simulink library "Generator_Lib"  (R2025a)
settings: Solver=ode45  StartTime=0.0  StopTime=10.0  RelTol=1e-3  EnableMultiTasking=on
undefined symbols (not defined in the file or in its folder): DiscIntNeverNeededParam, K, Lambda, radps2rpm, tau, WT_Params, x0
libraries: fl_lib x24, nesl_utility x16, ee_lib x14, simulink x1
(part 1 of 2)
Description:
  | Copyright 2009-2024 The MathWorks, Inc. MathWorks, Inc.
settings Model: Creator=smiller  LastModifiedBy=smiller
settings SolverCC: AlgebraicLoopSolver=TrustRegion
settings DataIOCC: LimitDataPoints=on  SaveFormat=Array  SignalLoggingSaveFormat=ModelDataLogs  ReturnWorkspaceOutputs=off
settings OptimizationCC: ReuseModelBlockBuffer=off  ExpressionDepthLimit=2147483647.0  LifeSpan=inf
settings DebuggingCC: UnderspecifiedInitializationDetection=Classic  MergeDetectMultiDrivingBlocksExec=none  SolverPrmCheckMsg=warning  FcnCallInpInsideContextMsg=warning  UnconnectedInputMsg=warning  UnconnectedOutputMsg=warning  UnconnectedLineMsg=warning  AllowSymbolicDim=off  StateNameClashWarn=warning  PregeneratedLibrarySubsystemCodeDiagnostic=none  SFUnexpectedBacktrackingDiag=warning  SFNoUnconditionalDefaultTransitionDiag=warning  SFExecutionAtInitializationDiag=none  ArithmeticOperatorsInVariantConditions=warning
settings HardwareCC: ProdBitPerPointer=32.0  ProdBitPerSizeT=32.0  ProdBitPerPtrDiffT=32.0  ProdLargestAtomicFloat=None  ProdIntDivRoundTo=Undefined  ProdEndianess=Unspecified  ProdWordSize=32.0  ProdHWDeviceType=32-bit Generic
settings ModelReferenceCC: EnableRefExpFcnMdlSchedulingChecks=on  PropagateSignalLabelsOutOfModel=off
settings SFSimCC: SimUseLocalCustomCode=off  CustomCodeUndefinedFunction=UseInterfaceOnly
settings RTWCC: RTWUseLocalCustomCode=off  GPUComputeCapability=3.5  DLArmComputeVersion=19.05
settings CodeAppCC: StateflowObjectComments=on
settings GRTTargetCC: TargetLangStandard=C89/C90 (ANSI)  CombineOutputUpdateFcns=off  GRTInterface=on
settings ConfigComp: CovMetricSettings=dw  CovSaveCumulativeToWorkspaceVar=on  CovSaveSingleToWorkspaceVar=on  CovExternalEMLEnable=off  CovSFcnEnable=off

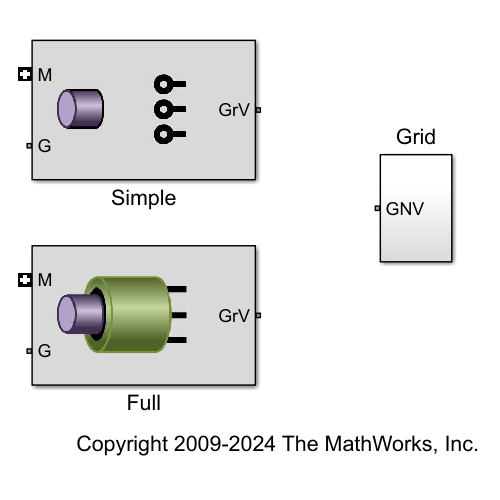
[thumbnail: Simulink's stored preview of the top-level diagram]
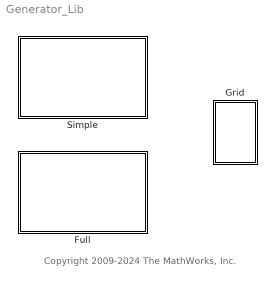
== system Generator_Lib ==
  note: Copyright 2009-2024 The MathWorks, Inc.
  Full : Subsystem  VariantControl=Full
      mask Display: image('Generator_Full_IMAGE.jpg');
  Grid : Subsystem
  Simple : Subsystem  VariantControl=Simple
      mask Display: image('Generator_Simple_IMAGE.jpg');

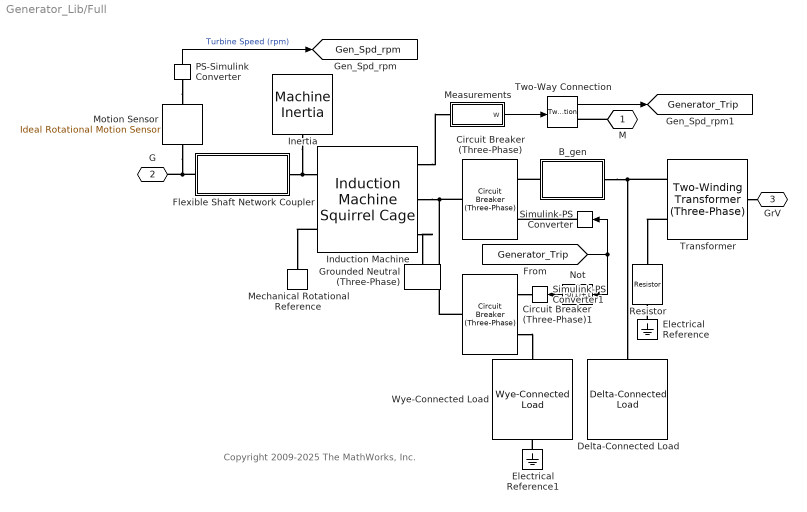
== system Generator_Lib/Full ==
  note: Copyright 2009-2025 The MathWorks, Inc.
  "B_gen " : Subsystem  mask{volt_meas=Phase-to-Ground (Phase Voltage), meas_units=PU, Vnom=WT_Params.Generator.voltage, Pnom=WT_Params.Generator.nominal_power}
      mask prompts: volt_meas "Voltage Measurement"; meas_units "Measurement Units"; Vnom "Nominal Voltage (Vrms)"; Pnom "Nominal Power (VA)"
      mask init:
      | volt_meas  = get_param(gcb,'volt_meas');
      | meas_units = get_param(gcb,'meas_units');
      | 
      | path_CV = [gcb,'/current_voltage'];
      | 
      | switch volt_meas
      | 
      |     case 'Phase-to-Ground (Phase Voltage)'
      | 
      |         set_param(path_CV,'vMeasurementType','ee.enum.vmeasurement.lg')
      | 
      |     case 'Line-to-Line (Line Voltage)'
      | 
      |         set_param(path_CV,'vMeasurementType','ee.enum.vmeasurement.ll')
      | 
      | end
      | 
      | switch meas_units
      | 
      |     case 'SI'
      | 
      |         set_param(path_CV,'outputUnit','ee.enum.unit.si')
      |         
      | 
      |     case 'PU'
      | 
      |         set_param(path_CV,'outputUnit','ee.enum.unit.pu')
      |       
      | 
      | end
      mask TypeOptions volt_meas: Phase-to-Ground (Phase Voltage) | Line-to-Line (Line Voltage)
      mask TypeOptions meas_units: SI | PU
      mask Callback meas_units:
      | meas_units = get_param(gcb,'meas_units');
      | 
      | switch meas_units
      | 
      |     case 'SI'
      | 
      |         set_param(gcb,'MaskVisibilities',{'on','on','off','off'})
      | 
      | 
      |     case 'PU'
      | 
      |         set_param(gcb,'MaskVisibilities',{'on','on','on','on'})
      | 
      | 
      | end
      mask DialogControl Container1 Prompt: Voltage and Current Measurement
      mask DialogControl Container2 Prompt: The block represents an ideal three-phase voltage and current sensor.
  Circuit Breaker (Three-Phase) : ee_lib/Switches & Breakers/Circuit Breaker (Three-Phase)  R_closed=WT_Params.Generator.Breakers.ron Ohm  G_open=1/WT_Params.Generator.Breakers.rp 1/Ohm  threshold=0.5 V  breaker_behavior=ee.enum.switches.breakerBehavior.zeroCrossingEnable
      settings: InternalSimscapePortConfiguration="{\"Bottom\":[],\"Left\":[{\"id\":\"vT\",\"label\":\"vT\",\"type\":\"input\"},{\"id\":\"N1\",\"label\":\"~1\",\"type\":\"foundation.electrical.three_phase\"}],\"Right\":[{\"id\":\"N2\",\"label\":\"~2\",\"type\":\"foundation.electrical.three_phase\"}],\"Top\":[]}"
  Circuit Breaker (Three-Phase)1 : ee_lib/Switches & Breakers/Circuit Breaker (Three-Phase)  R_closed=WT_Params.Generator.Breakers.ron Ohm  G_open=1/WT_Params.Generator.Breakers.rp 1/Ohm  threshold=0.5 V  breaker_behavior=ee.enum.switches.breakerBehavior.zeroCrossingEnable
      settings: InternalSimscapePortConfiguration="{\"Bottom\":[],\"Left\":[{\"id\":\"vT\",\"label\":\"vT\",\"type\":\"input\"},{\"id\":\"N1\",\"label\":\"~1\",\"type\":\"foundation.electrical.three_phase\"}],\"Right\":[{\"id\":\"N2\",\"label\":\"~2\",\"type\":\"foundation.electrical.three_phase\"}],\"Top\":[]}"
  Delta-Connected Load : ee_lib/Passive/RLC Assemblies/Delta-Connected Load  port_option=ee.enum.threePhasePort.composite  parameterization=ee.enum.rlc.parameterization.ratedpower  component_structure=ee.enum.rlc.structure.R  component_structure_PQ=ee.enum.rlc.structure.C  R=1 Ohm  L=1e-3 H  C=1e-6 F  VRated=WT_Params.Generator.voltage V  FRated=WT_Params.Generator.frequency Hz  P=1e3 W  Qpos=1e2 A*V  Qneg=-200e3 A*V  R_parasitic=0 Ohm  G_parasitic=0 1/Ohm  R_parasitic_PQ=0 Ohm  G_parasitic_PQ=0 1/Ohm  Vmag0=24e3 V  Vang0=0 deg  Freq0=60 Hz  IL_specify=off  IL_priority=High  IL=[0, 0, 0] A  IL_nominal_specify=off  IL_nominal_value=1  IL_nominal_unit=A  VC_specify=off  VC_priority=High  VC=[0, 0, 0] V  VC_nominal_specify=off  VC_nominal_value=1  VC_nominal_unit=V
      settings: InternalSimscapePortConfiguration="{\"Bottom\":[],\"Left\":[{\"id\":\"N\",\"label\":\"~\",\"type\":\"foundation.electrical.three_phase\"}],\"Right\":[],\"Top\":[]}"
  Electrical Reference : fl_lib/Electrical/Electrical Elements/Electrical Reference
  Electrical Reference1 : fl_lib/Electrical/Electrical Elements/Electrical Reference
  Flexible Shaft Network Coupler : Subsystem  mask(Network Coupler (Flexible Shaft)){}
      mask init:
      | % Icon
      | key = 'Simscape.NetworkCouplers.FlexibleShaft';
      | foundation.internal.couplers.updateIcon(gcb,'flexibleShaft.svg',key)
      settings: OpenFcn=open_system(gcbh,'force')
      mask Help: web([docroot '/simscape/ref/networkcouplerflexibleshaft.html'])
      mask Display:
      | color('red');
      | port_label('LConn', 1,'1')
      | port_label('RConn', 1,'2')
  Grounded Neutral (Three-Phase) : ee_lib/Connectors & References/Grounded Neutral (Three-Phase)
  Induction Machine : ee_lib/Electromechanical/Asynchronous/Induction Machine Squirrel Cage  port_option=ee.enum.threePhasePort.composite  SRated=WT_Params.Generator.nominal_power A*V  VRated=WT_Params.Generator.voltage V  FRated=WT_Params.Generator.frequency Hz  nPolePairs=3  param_unit=ee.enum.unit.pu  squirrel_cage=ee.enum.squirrelcage.Single  zero_sequence=ee.enum.park.zerosequence.exclude  initialization_option=ee.enum.asm.initialization.fluxvariables  Rs=Rs Ohm  Xls=Xls Ohm  pu_Rs=WT_Params.Generator.Stator.resistance  pu_Lls=WT_Params.Generator.Stator.inductance  Rrd=Rrp Ohm  Xlrd=Xlrp Ohm  pu_Rrd=WT_Params.Generator.Rotor.resistance  pu_Llrd=WT_Params.Generator.Rotor.inductance  Rrd1=0.28 Ohm  Xlrd1=0.82 Ohm  Rrd2=0.28 Ohm  Xlrd2=0.82 Ohm  pu_Rrd1=0.0290  pu_Llrd1=0.0848  pu_Rrd2=0.0290  pu_Llrd2=0.0848  Xm=Xm Ohm  pu_Lm=WT_Params.Generator.mutual_inductance  X0=0.4 Ohm  pu_L0=0.0413  saturation_option=ee.enum.saturation.exclude  saturation_i=[0, 4, 9, 18, 25, 34, 50, 68, 95, 120] A  saturation_v=[0, 88, 154, 198, 220, 242, 264, 286, 308, 327] V  pu_saturation_i=[0, .176, .396, .792, 1.1, 1.496, 2.2, 2.992, 4.18, 5.28]  pu_saturation_v=[0, .4, .7, .9, 1, 1.1, 1.2, 1.3, 1.4, 1.4864]  connection_option=ee.enum.Connection.delta  angular_position_specify=off  angular_position_priority=None  angular_position=0 deg  angular_position_nominal_specify=off  angular_position_nominal_value=1  angular_position_nominal_unit=deg  pu_psids_specify=off  pu_psids_priority=None  pu_psids=0  pu_psids_nominal_specify=off  pu_psids_nominal_value=1  pu_psids_nominal_unit=1  pu_psiqs_specify=off  pu_psiqs_priority=None  pu_psiqs=0  pu_psiqs_nominal_specify=off  pu_psiqs_nominal_value=1  pu_psiqs_nominal_unit=1  pu_psi0s_specify=off  pu_psi0s_priority=None  pu_psi0s=0  pu_psi0s_nominal_specify=off  pu_psi0s_nominal_value=1  pu_psi0s_nominal_unit=1  pu_psidr_specify=off  pu_psidr_priority=None  pu_psidr=0  pu_psidr_nominal_specify=off  pu_psidr_nominal_value=1  pu_psidr_nominal_unit=1  pu_psiqr_specify=off  pu_psiqr_priority=None  pu_psiqr=0  pu_psiqr_nominal_specify=off  pu_psiqr_nominal_value=1  pu_psiqr_nominal_unit=1  pu_psidr1_specify=off  pu_psidr1_priority=None  pu_psidr1=0  pu_psidr1_nominal_specify=off  pu_psidr1_nominal_value=1  pu_psidr1_nominal_unit=1  pu_psiqr1_specify=off  pu_psiqr1_priority=None  pu_psiqr1=0  pu_psiqr1_nominal_specify=off  pu_psiqr1_nominal_value=1  pu_psiqr1_nominal_unit=1  pu_psidr2_specify=off  pu_psidr2_priority=None  pu_psidr2=0  pu_psidr2_nominal_specify=off  pu_psidr2_nominal_value=1  pu_psidr2_nominal_unit=1  pu_psiqr2_specify=off  pu_psiqr2_priority=None  pu_psiqr2=0  pu_psiqr2_nominal_specify=off  pu_psiqr2_nominal_value=1  pu_psiqr2_nominal_unit=1  psids_specify=off  psids_priority=None  psids=0 Wb  psids_nominal_specify=off  psids_nominal_value=1  psids_nominal_unit=Wb  psiqs_specify=off  psiqs_priority=None  psiqs=0 Wb  psiqs_nominal_specify=off  psiqs_nominal_value=1  psiqs_nominal_unit=Wb  psi0s_specify=off  psi0s_priority=None  psi0s=0 Wb  psi0s_nominal_specify=off  psi0s_nominal_value=1  psi0s_nominal_unit=Wb  psidr_specify=off  psidr_priority=None  psidr=0 Wb  psidr_nominal_specify=off  psidr_nominal_value=1  psidr_nominal_unit=Wb  psiqr_specify=off  psiqr_priority=None  psiqr=0 Wb  psiqr_nominal_specify=off  psiqr_nominal_value=1  psiqr_nominal_unit=Wb  psidr1_specify=off  psidr1_priority=None  psidr1=0 Wb  psidr1_nominal_specify=off  psidr1_nominal_value=1  psidr1_nominal_unit=Wb  psiqr1_specify=off  psiqr1_priority=None  psiqr1=0 Wb  psiqr1_nominal_specify=off  psiqr1_nominal_value=1  psiqr1_nominal_unit=Wb  psidr2_specify=off  psidr2_priority=None  psidr2=0 Wb  psidr2_nominal_specify=off  psidr2_nominal_value=1  psidr2_nominal_unit=Wb  psiqr2_specify=off  psiqr2_priority=None  psiqr2=0 Wb  psiqr2_nominal_specify=off  psiqr2_nominal_value=1  psiqr2_nominal_unit=Wb  slip_specify=off  slip_priority=None  slip=0  slip_nominal_specify=off  slip_nominal_value=1  slip_nominal_unit=1  real_power_generated_specify=off  real_power_generated_priority=None  real_power_generated=0 W  real_power_generated_nominal_specify=off  real_power_generated_nominal_value=1  real_power_generated_nominal_unit=W  mechanical_power_consumed_specify=off  mechanical_power_consumed_priority=None  mechanical_power_consumed=0 W  mechanical_power_consumed_nominal_specify=off  mechanical_power_consumed_nominal_value=1  mechanical_power_consumed_nominal_unit=W  Tmeas=298.15 K  alpha=3.93e-3 1/K  alpha_cage=4.4e-3 1/K  stator_thermal_mass=100 J/K  rotor_thermal_mass=200 J/K  temperatureA_specify=off  temperatureA_priority=High  temperatureA=25 degC  temperatureA_nominal_specify=off  temperatureA_nominal_value=1  temperatureA_nominal_unit=degC  temperatureB_specify=off  temperatureB_priority=High  temperatureB=25 degC  temperatureB_nominal_specify=off  temperatureB_nominal_value=1  temperatureB_nominal_unit=degC  temperatureC_specify=off  temperatureC_priority=High  temperatureC=25 degC  temperatureC_nominal_specify=off  temperatureC_nominal_value=1  temperatureC_nominal_unit=degC  temperatureR_specify=off  temperatureR_priority=High  temperatureR=25 degC  temperatureR_nominal_specify=off  temperatureR_nominal_value=1  temperatureR_nominal_unit=degC
      settings: InternalSimscapePortConfiguration="{\"Bottom\":[],\"Left\":[{\"id\":\"R\",\"label\":\"R\",\"type\":\"foundation.mechanical.rotational.rotational\"},{\"id\":\"C\",\"label\":\"C\",\"type\":\"foundation.mechanical.rotational.rotational\"}],\"Right\":[{\"id\":\"pu_output\",\"label\":\"pu\",\"type\":\"output\"},{\"id\":\"N1\",\"label\":\"~1\",\"type\":\"foundation.electrical.three_phase\"},{\"id\":\"N2\",\"label\":\"~2\",\"type\":\"foundation.electrical.three_phase\"}],\"Top\":[]}"
  Inertia : ee_lib/Electromechanical/Mechanical/Machine Inertia  SRated=WT_Params.Generator.nominal_power A*V  FRated=WT_Params.Generator.frequency Hz  nPolePairs=3  inertia_option=1  J=3 kg*m^2  H=3.525 W*s/(A*V)  damper_option=2  D=39.0509 N*m*s/rad  pu_D=0  initialization_option=2  fMechanical0=60 Hz  fElectrical0=0 Hz
      settings: InternalSimscapePortConfiguration="{\"Bottom\":[],\"Left\":[{\"id\":\"R\",\"label\":\"R\",\"type\":\"foundation.mechanical.rotational.rotational\"}],\"Right\":[],\"Top\":[]}"
  Measurements : Subsystem
  Mechanical Rotational Reference : fl_lib/Mechanical/Rotational Elements/Mechanical Rotational Reference
  Motion Sensor : fl_lib/Mechanical/Mechanical Sensors/Ideal Rotational Motion Sensor  reference=foundation.enum.MeasurementReference.absolute  acceleration_port=false  velocity_port=true  position_port=false  wrap_angle=simscape.enum.onoff.off  offset=0 rad
      settings: InternalSimscapePortConfiguration="{\"Bottom\":[],\"Left\":[{\"id\":\"R\",\"label\":\"R\",\"type\":\"foundation.mechanical.rotational.rotational\"}],\"Right\":[{\"id\":\"W\",\"label\":\"W\",\"type\":\"output\"}],\"Top\":[]}"
  Not : Fcn  Expr=-u(1)+1
  PS-Simulink Converter : nesl_utility/PS-Simulink Converter  PhysicalDomain=network_engine_domain  SubClassName=ps_output  LeftPortType=input  RightPortType=output  PseudoPeriodic=off  Frequencies=[]  VectorFormat=1-D array  Unit=rpm  AffineConversion=off
  Resistor : fl_lib/Electrical/Electrical Elements/Resistor  R=10 Ohm  i_specify=off  i_priority=None  i=0 A  i_nominal_specify=off  i_nominal_value=1  i_nominal_unit=A  v_specify=off  v_priority=None  v=0 V  v_nominal_specify=off  v_nominal_value=1  v_nominal_unit=V
  Simulink-PS Converter : nesl_utility/Simulink-PS Converter  PhysicalDomain=network_engine_domain  SubClassName=ps_input  LeftPortType=input  RightPortType=output  PseudoPeriodic=off  Frequencies=[]  NoiseDistribution=none  NoiseParameters=[]  Unit=1  AffineConversion=off  FilteringAndDerivatives=provide  SimscapeFilterOrder=1  InputFilterTimeConstant=0.001  UdotUserProvided=0
  Simulink-PS Converter1 : nesl_utility/Simulink-PS Converter  PhysicalDomain=network_engine_domain  SubClassName=ps_input  LeftPortType=input  RightPortType=output  PseudoPeriodic=off  Frequencies=[]  NoiseDistribution=none  NoiseParameters=[]  Unit=1  AffineConversion=off  FilteringAndDerivatives=provide  SimscapeFilterOrder=1  InputFilterTimeConstant=0.001  UdotUserProvided=0
  Transformer : ee_lib/Passive/Transformers/Two-Winding Transformer (Three-Phase)  SRated=2e6 A*V  FRated=60 Hz  Winding1Connection=ee.enum.windingconnection.Yg  VRated1=WT_Params.Grid.voltage V  Winding2Connection=ee.enum.windingconnection.Yn  VRated2=WT_Params.Generator.voltage V  CoreType=ee.enum.coretype.threelimb  pu_Rw1=0.025/30  pu_Rw2=0.025/30  leakage_reactance_option=ee.enum.transformer_leakage.include  pu_Xl1=0.025  pu_Xl2=0.025  magnetizing_resistance_option=ee.enum.transformer_magnetizingResistance.include  pu_Rm=500  magnetizing_reactance_option=ee.enum.transformer_magnetizingReactance.include  saturation_option=ee.enum.transformer_saturation.exclude  pu_Xm=500  current_data=[0, .002, 1, 2]  magnetic_flux_data=[0, 1.2, 1.5, 1.51]  pu_X0=0.5  i1_specify=off  i1_priority=None  i1=[0, 0, 0] A  i1_nominal_specify=off  i1_nominal_value=1  i1_nominal_unit=A  i2_specify=off  i2_priority=None  i2=[0, 0, 0] A  i2_nominal_specify=off  i2_nominal_value=1  i2_nominal_unit=A  phi_specify=off  phi_priority=None  phi=[0, 0, 0]  phi_nominal_specify=off  phi_nominal_value=1  phi_nominal_unit=1  power_dissipated_specify=off  power_dissipated_priority=None  power_dissipated=0 W  power_dissipated_nominal_specify=off  power_dissipated_nominal_value=1  power_dissipated_nominal_unit=W
      settings: InternalSimscapePortConfiguration="{\"Bottom\":[],\"Left\":[{\"id\":\"N1\",\"label\":\"~1\",\"type\":\"foundation.electrical.three_phase\"}],\"Right\":[{\"id\":\"N2\",\"label\":\"~2\",\"type\":\"foundation.electrical.three_phase\"},{\"id\":\"n2\",\"label\":\"n2\",\"type\":\"foundation.electrical.electrical\"}],\"Top\":[]}"
  Two-Way Connection : TwoWayConnection
  Wye-Connected Load : ee_lib/Passive/RLC Assemblies/Wye-Connected Load  port_option=ee.enum.threePhasePort.composite  parameterization=ee.enum.rlc.parameterization.ratedpower  component_structure=ee.enum.rlc.structure.R  component_structure_PQ=ee.enum.rlc.structure.R  R=1 Ohm  L=1e-3 H  C=1e-6 F  VRated=WT_Params.Generator.voltage V  FRated=60 Hz  P=WT_Params.Generator.nominal_power W  Qpos=1e2 A*V  Qneg=-1e2 A*V  R_parasitic=0 Ohm  G_parasitic=0 1/Ohm  R_parasitic_PQ=0 Ohm  G_parasitic_PQ=0 1/Ohm  Vmag0=24e3 V  Vang0=0 deg  Freq0=60 Hz  IL_specify=off  IL_priority=High  IL=[0, 0, 0] A  IL_nominal_specify=off  IL_nominal_value=1  IL_nominal_unit=A  VC_specify=off  VC_priority=High  VC=[0, 0, 0] V  VC_nominal_specify=off  VC_nominal_value=1  VC_nominal_unit=V
  M : PMIOPort  Tag=PMCPort  Side=Left
  G : PMIOPort  Port=2  Side=Left
  GrV : PMIOPort  Port=3  Side=Right
  tag scope: Gen_Spd_rpm=global, Generator_Trip=global
  wires:
  PS-Simulink Converter/1 -> [Gen_Spd_rpm]  "Turbine Speed (rpm)"
  Two-Way Connection/1 -> [Generator_Trip]
  Not/1 -> Simulink-PS Converter1/1
  [Generator_Trip] -> Not/1, Simulink-PS Converter/1
  Measurements/1(w) -> Two-Way Connection/1
  connections:
  Flexible Shaft Network Coupler/LConn1 -- G/RConn1 -- Motion Sensor/LConn1
  M/RConn1 -- Two-Way Connection/RConn1
  Transformer/LConn1 -- GrV/RConn1
  Electrical Reference/LConn1 -- Resistor/LConn1
  Transformer/RConn2 -- Resistor/RConn1
  Transformer/RConn1 -- "B_gen "/RConn1 -- Delta-Connected Load/LConn1
  Circuit Breaker (Three-Phase)/RConn1 -- Circuit Breaker (Three-Phase)1/RConn1 -- Induction Machine/RConn2
  Electrical Reference1/LConn1 -- Wye-Connected Load/RConn1
  "B_gen "/LConn1 -- Circuit Breaker (Three-Phase)/LConn2
  Circuit Breaker (Three-Phase)1/LConn2 -- Wye-Connected Load/LConn1
  Simulink-PS Converter/RConn1 -- Circuit Breaker (Three-Phase)/LConn1
  Circuit Breaker (Three-Phase)1/LConn1 -- Simulink-PS Converter1/RConn1
  PS-Simulink Converter/LConn1 -- Motion Sensor/RConn1
  Induction Machine/LConn2 -- Mechanical Rotational Reference/LConn1
  Flexible Shaft Network Coupler/RConn1 -- Inertia/LConn1 -- Induction Machine/LConn1
  Induction Machine/RConn3 -- Grounded Neutral (Three-Phase)/LConn1
  Induction Machine/RConn1 -- Measurements/LConn1

== system Generator_Lib/Grid ==
  note: Copyright 2009-2025 The MathWorks, Inc.
  Electrical Reference : fl_lib/Electrical/Electrical Elements/Electrical Reference
  Grid : ee_lib/Sources/Voltage Source (Three-Phase)  vline_rms=WT_Params.Grid.voltage V  shift=0 deg  freq=WT_Params.Grid.frequency Hz  impedance_option=0  SShortCircuit=1e6 A*V  XR=15  R=0.01 Ohm  L=3.97e-4 H  harmonic_option=0  harmonic_orders=[5, 7, 11, 13]  harmonic_ratios=[.1, .1, .1, .1]  G_parasitic=0 1/Ohm  I_specify=off  I_priority=None  I=[0, 0, 0] A  I_nominal_specify=off  I_nominal_value=1  I_nominal_unit=A
  Mutual RL Pos-Zero (SI) : Subsystem  mask{R1_L1=[0.1  1.0/(2*pi*60)]*WT_Params.Grid.voltage^2/2500e6, R0_L0=[0.3  3.0/(2*pi*60)]*WT_Params.Grid.voltage^2/2500e6, run_time=off}
      mask prompts: R1_L1 "Positive Sequence [R1(Ohm) L1(H)]"; R0_L0 "Zero Sequence [R0(Ohm) L0(H)]"; run_time "Set parameters to run-time (model does not recompile if parameters change value)"
      mask init:
      | maskObj = Simulink.Mask.get(gcbh);
      | workspaceObj = maskObj.getWorkspace();
      | 
      | R1_L1 = workspaceObj.get('R1_L1');
      | R0_L0 = workspaceObj.get('R0_L0');
      | 
      | R1_si = R1_L1(1);
      | L1_si = R1_L1(2);
      | R0_si = R0_L0(1);
      | L0_si = R0_L0(2);
      | 
      | Rs_si = (2*R1_si + R0_si)/3;
      | Rm_si = (R0_si - R1_si)/3;
      | 
      | Ls_si = (2*L1_si + L0_si)/3;
      | Lm_si = (L0_si - L1_si)/3;
      mask Callback run_time:
      | run_time = get_param(gcb,'run_time');
      | 
      | path_coupled = [gcb,'/Coupled'];
      | 
      | switch run_time
      |     case 'off'
      |         pcr = 'compiletime';
      |     case 'on'
      |         pcr = 'runtime';
      | end
      | 
      | set_param(path_coupled,'R_conf',pcr)
      | set_param(path_coupled,'Rm_conf',pcr)
      | set_param(path_coupled,'L_conf',pcr)
      | set_param(path_coupled,'Lm_conf',pcr)
      mask DialogControl DescGroupVar Prompt: Mutual RL Pos-Zero
      mask DialogControl DescTextVar Prompt: Define mutual RL with positive and zero sequence values
      mask DialogControl Container5 Prompt: Parameters
      mask Display: disp('Mutual RL\n Pos-Zero\n(SI)')
  Pi-Section Pos-Zero (SI) : Subsystem  mask{length=1, Fnom=WT_Params.Grid.frequency, R1_L1_C1=[0.1153 1.05e-3 11.33e-9], R0_L0_C0=[0.413 3.32e-3 5.01e-9], run_time=off}
      mask prompts: length "Line Length (km)"; Fnom "Nominal Frequency (Hz)"; R1_L1_C1 "Positive Sequence [R1(Ohm/km) L1(H/km) C1(F/km)]"; R0_L0_C0 "Zero Sequence [R0(Ohm/km) L0(H/km) C0(F/km)]"; run_time "Set parameters to run-time (model does not recompile if parameters change value)"
      mask init:
      | maskObj = Simulink.Mask.get(gcbh);
      | workspaceObj = maskObj.getWorkspace();
      | 
      | R1_L1_C1 = workspaceObj.get('R1_L1_C1');
      | R0_L0_C0 = workspaceObj.get('R0_L0_C0');
      | 
      | R1_si = R1_L1_C1(1);
      | L1_si = R1_L1_C1(2);
      | C1_si = R1_L1_C1(3);
      | R0_si = R0_L0_C0(1);
      | L0_si = R0_L0_C0(2);
      | C0_si = R0_L0_C0(3);
      | 
      | Rs_si = (2*R1_si + R0_si)/3;
      | Rm_si = (R0_si - R1_si)/3;
      | 
      | Ls_si = (2*L1_si + L0_si)/3;
      | Lm_si = (L0_si - L1_si)/3;
      | 
      | Cl_si = (C1_si-C0_si)/3;
      | Cg_si = C0_si;
      mask Callback run_time:
      | run_time = get_param(gcb,'run_time');
      | 
      | path_line = [gcb,'/line'];
      | 
      | switch run_time
      |     case 'off'
      |         pcr = 'compiletime';
      |     case 'on'
      |         pcr = 'runtime';
      | end
      | 
      | set_param(path_line,'freq_conf',pcr)
      | set_param(path_line,'length_conf',pcr)
      | set_param(path_line,'R_conf',pcr)
      | set_param(path_line,'L_conf',pcr)
      | set_param(path_line,'Rm_conf',pcr)
      | set_param(path_line,'M_conf',pcr)
      | set_param(path_line,'Cg_conf',pcr)
      | set_param(path_line,'Cl_conf',pcr)
      mask DialogControl DescGroupVar Prompt: Pi-Section Pos-Zero (SI)
      mask DialogControl DescTextVar Prompt: Define pi-section line with positive and zero sequence values
      mask DialogControl Container5 Prompt: Parameters
      mask Display: disp('Pi-Section\nPos-Zero\n(SI)')
  GNV : PMIOPort  Side=Right
  connections:
  Grid/RConn1 -- Mutual RL Pos-Zero (SI)/RConn1
  Electrical Reference/LConn1 -- Grid/LConn1
  Mutual RL Pos-Zero (SI)/LConn1 -- Pi-Section Pos-Zero (SI)/RConn1
  GNV/RConn1 -- Pi-Section Pos-Zero (SI)/LConn1

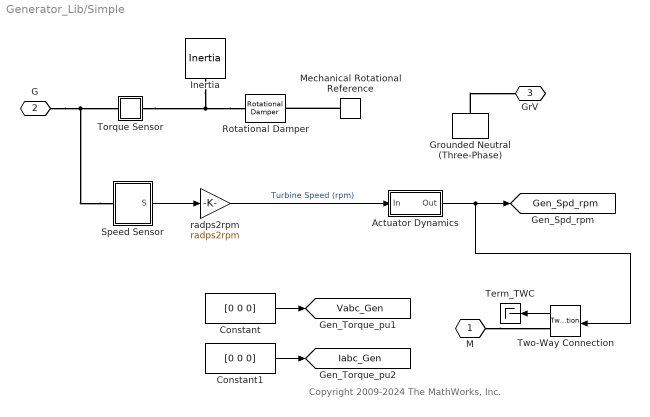
== system Generator_Lib/Simple ==
  note: Copyright 2009-2024 The MathWorks, Inc.
  Actuator Dynamics : Subsystem  mask(First-order lag supporting vector signals){b=WT_Params.Generator.generator_time_constant, x_initial=0}
      mask prompts: b "Filter time constant"; x_initial "Initial output"
      mask help: Models a lag of the form 1/(b*s+1) where s is the Laplace operator.
  Constant : Constant  Value=[0 0 0]  OutDataTypeStr=Inherit: Inherit via back propagation
  Constant1 : Constant  Value=[0 0 0]  OutDataTypeStr=Inherit: Inherit via back propagation
  Grounded Neutral (Three-Phase) : ee_lib/Connectors & References/Grounded Neutral (Three-Phase)
  Inertia : fl_lib/Mechanical/Rotational Elements/Inertia  inertia=WT_Params.Generator.Simple.inertia kg*m^2  num_ports=foundation.enum.numPorts2.one  w_specify=on  w_priority=High  w=0 rad/s  w_nominal_specify=off  w_nominal_value=1  w_nominal_unit=rad/s  t_specify=off  t_priority=High  t=0 N*m  t_nominal_specify=off  t_nominal_value=1  t_nominal_unit=N*m
  Mechanical Rotational Reference : fl_lib/Mechanical/Rotational Elements/Mechanical Rotational Reference
  Rotational Damper : fl_lib/Mechanical/Rotational Elements/Rotational Damper  D=WT_Params.Generator.Simple.damping N*m/(rad/s)  w_specify=off  w_priority=High  w=0 rad/s  w_nominal_specify=off  w_nominal_value=1  w_nominal_unit=rad/s  t_specify=off  t_priority=High  t=0 N*m  t_nominal_specify=off  t_nominal_value=1  t_nominal_unit=N*m
  Speed Sensor : Subsystem
      mask Display:
      | plot([149.600878633536;150.016472378793;150.47508104106;150.972287968219;151.50330478576;152.063017511447;152.646035805762;153.246744883819;153.859359588817;154.477980106257;155.096648782383;155.709407499646;156.310355056631;156.893703999851;157.453836360095;157.985357756531;158.483149347555;158.942417128023;159.358738098149;159.728102859405;160.046954227227;160.312221488639;160.521349974904;160.672325664379;160.763694578642;160.794576785101;160.764674871227;160.674276808796;160.524253180566;160.316048796087;160.051668777399;159.733659248606;159.365082815313;158.949489070056;158.490880407788;157.993673480629;157.462656663088;156.908284800231], [156.971389291536;157.430657072004;157.84697804213;158.216342803387;158.535194171208;158.80046143262;159.009589918885;159.16056560836;159.251934522623;159.282816729083;159.252914815208;159.162516752777;159.012493124547;158.804288740068;158.53990872138;158.221899192587;157.853322759294;157.437729014037;156.979120351769;156.48191342461;155.950896607069;155.391183881382;154.808165587067;154.20745650901;153.594841804012;152.976221286573;152.357552610446;151.744793893183;151.143846336199;150.560497392978;150.000365032735;149.468843636298;148.971052045274;148.511784264806;148.095463294681;147.726098533424;147.407247165603;147.144199990631])
      | plot([152.057635404444;152.93604260309;153.834625296826;154.744729643097;155.657590839533;156.564417533794;157.45647648909;158.325176690034;159.162152078811;159.959342124889;160.709069452336;161.404113777147;162.037781442523;162.603969882449;163.097226392739;163.512800643557;163.846690427691;164.095680203997;164.257372064819;164.330208829146;164.313489039122;164.27939575172], [142.228020686971;141.979030910664;141.817339049842;141.744502285515;141.761222075539;141.867337399197;142.061826307913;142.342815767178;142.707599694895;143.152665022428;143.673725527376;144.265763112236;144.923076131425;145.639334301243;146.40763966397;147.220593018964;148.070365181011;148.948772379657;149.847355073393;150.757459419663;151.6703206161;152.055850472277])
      | plot([116.468514315784;116.438789536125;116.349901463023;116.202706137216;115.998621130155;115.739611892022;115.42817282337;115.067303252679;114.660478551187;114.211616663162;113.725040373958;113.205435679231;112.657806656235;112.087427271827;111.499790591278;110.900555877058;110.29549408704;109.690432297022;109.091197582803;108.503560902254;107.933181517846;107.38555249485;106.865947800123;106.379371510919;105.930509622894;105.523684921402;105.162815350711;104.851376282059;104.592367043926;104.388282036865;104.241086711057;104.152198637956;104.122473858297;104.152198637956;104.241086711057;104.388282036865;104.592367043926;104.851376282059;105.162815350711;105.523684921402;105.930509622894;106.379371510919;106.865947800123;107.38555249485;107.933181517846;108.503560902254;109.091197582803;109.690432297022;110.29549408704;110.900555877058;111.499790591278;112.087427271827;112.657806656235;113.205435679231;113.725040373958;114.211616663162;114.660478551187;115.067303252679;115.42817282337;115.739611892022;115.998621130155;116.202706137216;116.349901463023;116.438789536125;116.468514315784;116.468514315784], [111.618284136057;111.013222346039;110.413987631819;109.826350951271;109.255971566862;108.708342543866;108.188737849139;107.702161559936;107.253299671911;106.846474970419;106.485605399728;106.174166331075;105.915157092943;105.711072085881;105.563876760074;105.474988686973;105.445263907313;105.474988686973;105.563876760074;105.711072085881;105.915157092943;106.174166331075;106.485605399728;106.846474970419;107.253299671911;107.702161559936;108.188737849139;108.708342543866;109.255971566862;109.826350951271;110.413987631819;111.013222346039;111.618284136057;112.223345926075;112.822580640295;113.410217320843;113.980596705252;114.528225728247;115.047830422975;115.534406712178;115.983268600203;116.390093301695;116.750962872386;117.062401941038;117.321411179171;117.525496186232;117.67269151204;117.761579585141;117.7913043648;117.761579585141;117.67269151204;117.525496186232;117.321411179171;117.062401941038;116.750962872386;116.390093301695;115.983268600203;115.534406712178;115.047830422975;114.528225728247;113.980596705252;113.410217320843;112.822580640295;112.223345926075;111.618284136057;111.618284136057])
      | plot([239.23602886498;238.828071429858;237.608127977604;235.587947230552;232.78698463364;229.232214987837;224.957872668068;220.005121927465;214.421660463109;208.261260061133;201.583248745024;194.451939414329;186.936010476274;179.107844435155;171.042830809261;162.818640088593;154.514475725591;146.210311362589;137.986120641921;129.921107016027;122.092940974909;114.577012036853;107.445702706158;100.76769139005;94.607290988073;89.0238295237172;84.0710787831142;79.7967364633452;76.2419668175427;73.4410042206305;71.4208234735788;70.2008800213248;69.7929225862026;70.2008800213248;71.4208234735788;73.4410042206306;76.2419668175428;79.7967364633454;84.0710787831144;89.0238295237174;94.6072909880733;100.76769139005;107.445702706159;114.577012036853;122.092940974909;129.921107016027;137.986120641921;146.210311362589;154.514475725591;162.818640088593;171.042830809261;179.107844435155;186.936010476274;194.451939414329;201.583248745024;208.261260061133;214.421660463109;220.005121927465;224.957872668068;229.232214987837;232.78698463364;235.587947230552;237.608127977604;238.828071429858;239.23602886498;239.23602886498], [155.774275772274;147.47628550917;139.258209428443;131.199192095207;123.376846251889;115.866505365088;108.740498123116;102.067451871182;95.9116316925529;90.3323215006612;85.3832531026163;81.1120887325275;77.5599620381344;74.7610819412943;72.742403187363;71.5233667562631;71.1157126352191;71.5233667562631;72.742403187363;74.7610819412943;77.5599620381345;81.1120887325275;85.3832531026164;90.3323215006612;95.9116316925529;102.067451871182;108.740498123116;115.866505365089;123.376846251889;131.199192095207;139.258209428443;147.47628550917;155.774275772274;164.072266035377;172.290342116104;180.34935944934;188.171705292658;195.682046179459;202.808053421432;209.481099673365;215.636919851994;221.216230043886;226.165298441931;230.43646281202;233.988589506413;236.787469603253;238.806148357184;240.025184788284;240.432838909328;240.025184788284;238.806148357184;236.787469603253;233.988589506413;230.43646281202;226.165298441931;221.216230043886;215.636919851994;209.481099673365;202.808053421432;195.682046179459;188.171705292658;180.34935944934;172.290342116105;164.072266035378;155.774275772274;155.774275772274])
      | plot([252.715889364481;252.243022716633;250.828976737403;248.487369462568;245.240751850236;241.120390602797;236.165967051481;230.425195003451;223.953361231755;216.812793033479;209.072257983804;200.806301666664;192.094529760025;183.020841389688;173.672621134841;164.139897466795;154.514475725591;144.889053984387;135.356330316341;126.008110061494;116.934421691157;108.222649784518;99.9566934673787;92.2161584177032;85.075590219427;78.6037564477313;72.8629843997015;67.9085608483856;63.7881996009461;60.5415819886144;58.199974713779;56.7859287345493;56.3130620867014;56.7859287345493;58.1999747137791;60.5415819886146;63.7881996009463;67.9085608483858;72.8629843997018;78.6037564477315;85.0755902194273;92.2161584177035;99.9566934673791;108.222649784519;116.934421691157;126.008110061494;135.356330316341;144.889053984387;154.514475725591;164.139897466796;173.672621134841;183.020841389688;192.094529760025;200.806301666664;209.072257983803;216.812793033479;223.953361231755;230.425195003451;236.165967051481;241.120390602797;245.240751850236;248.487369462568;250.828976737403;252.243022716633;252.715889364481;252.715889364481], [154.514475725591;144.895228084285;135.36861905618;126.026395093992;116.958526921455;108.252343066071;99.9916888376535;92.2561188521535;85.1201308772245;78.6524483779929;72.9153586725213;67.9641130708855;63.8463947748555;60.6018596625959;58.2617543808809;56.8486154228053;56.3760520890355;56.8486154228053;58.2617543808809;60.6018596625959;63.8463947748555;67.9641130708856;72.9153586725213;78.652448377993;85.1201308772246;92.2561188521536;99.9916888376536;108.252343066072;116.958526921455;126.026395093992;135.36861905618;144.895228084285;154.514475725591;164.133723366898;173.660332395002;183.002556357191;192.070424529728;200.776608385111;209.037262613529;216.772832599029;223.908820573958;230.37650307319;236.113592778661;241.064838380297;245.182556676327;248.427091788587;250.767197070302;252.180336028377;252.652899362147;252.180336028377;250.767197070301;248.427091788587;245.182556676327;241.064838380297;236.113592778661;230.37650307319;223.908820573958;216.772832599029;209.037262613529;200.776608385111;192.070424529728;183.002556357191;173.660332395002;164.133723366898;154.514475725592;154.514475725591])
      | plot([154.514475725591;129.948374815285;179.017586633563;154.514475725591], [240.369848906994;203.583687543869;203.583687543869;240.369848906994])
      | plot([105.382273904979;149.60125554353], [115.271704271436;156.971085816622])
      | plot([144.688035361469;144.688035361469], [152.057865634561;203.583687543869])
      | plot([164.277926087379;164.277926087379], [152.057865634561;203.583687543869])
      | plot([159.112745895982;159.616665914655], [149.60125554353;149.60125554353])
      | plot([115.208714269102;159.364705905318], [107.901873998344;149.60125554353])
      | plot([0;311.800511553884;311.800511553884;0;0], [311.800511553884;311.800511553884;0;0;311.800511553884])
      | ;
      | color('red');
      | port_label('LConn', 1,'R')
      | port_label('output', 1,'W')
  Term_TWC : Terminator
  Torque Sensor : Subsystem
      mask Display: disp('S');
  Two-Way Connection : TwoWayConnection
  radps2rpm : Gain  Gain=radps2rpm
  M : PMIOPort  Tag=PMCPort  Side=Left
  G : PMIOPort  Port=2  Side=Left
  GrV : PMIOPort  Port=3  Side=Right
  tag scope: Gen_Spd_rpm=global, Iabc_Gen=global, Vabc_Gen=global
  wires:
  Actuator Dynamics/1(Out) -> [Gen_Spd_rpm], Two-Way Connection/1
  Two-Way Connection/1 -> Term_TWC/1
  radps2rpm/1 -> Actuator Dynamics/1(In)  "Turbine Speed (rpm)"
  Speed Sensor/1(S) -> radps2rpm/1
  Constant/1 -> [Vabc_Gen]
  Constant1/1 -> [Iabc_Gen]
  connections:
  Rotational Damper/LConn1 -- Inertia/LConn1 -- Torque Sensor/RConn1
  Mechanical Rotational Reference/LConn1 -- Rotational Damper/RConn1
  Speed Sensor/LConn1 -- G/RConn1 -- Torque Sensor/LConn1
  M/RConn1 -- Two-Way Connection/RConn1
  Grounded Neutral (Three-Phase)/LConn1 -- GrV/RConn1

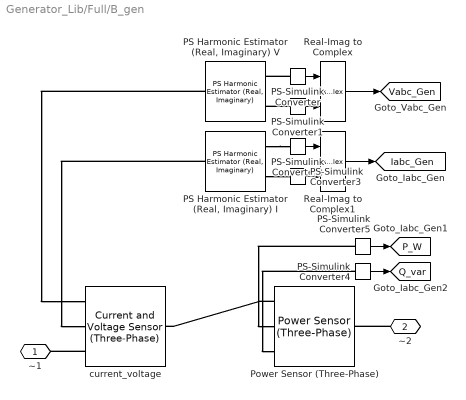
== system Generator_Lib/Full/B_gen  ==
  "PS Harmonic Estimator (Real, Imaginary) I" : fl_lib/Physical Signals/Periodic Operators/PS Harmonic Estimator (Real, Imaginary)  f0=60 Hz  n=1
      settings: InternalSimscapePortConfiguration="{\"Bottom\":[],\"Left\":[{\"id\":\"I\",\"label\":\"I\",\"type\":\"input\"}],\"Right\":[{\"id\":\"Re\",\"label\":\"Re\",\"type\":\"output\"},{\"id\":\"Im\",\"label\":\"Im\",\"type\":\"output\"}],\"Top\":[]}"
  "PS Harmonic Estimator (Real, Imaginary) V" : fl_lib/Physical Signals/Periodic Operators/PS Harmonic Estimator (Real, Imaginary)  f0=60 Hz  n=1
      settings: InternalSimscapePortConfiguration="{\"Bottom\":[],\"Left\":[{\"id\":\"I\",\"label\":\"I\",\"type\":\"input\"}],\"Right\":[{\"id\":\"Re\",\"label\":\"Re\",\"type\":\"output\"},{\"id\":\"Im\",\"label\":\"Im\",\"type\":\"output\"}],\"Top\":[]}"
  PS-Simulink Converter{,1..5} (6 alike) : nesl_utility/PS-Simulink Converter  PhysicalDomain=network_engine_domain  SubClassName=ps_output  LeftPortType=input  RightPortType=output  PseudoPeriodic=off  Frequencies=[]  VectorFormat=inherit  Unit=inherit  AffineConversion=off
  Power Sensor (Three-Phase) : ee_lib/Sensors & Transducers/Power Sensor (Three-Phase)  load_type=ee.enum.passive.type_balanced.balanced  f0=60 Hz  config=ee.enum.with_neutral.no  rho=1
      settings: InternalSimscapePortConfiguration="{\"Bottom\":[],\"Left\":[{\"id\":\"N1\",\"label\":\"~1\",\"type\":\"foundation.electrical.three_phase\"}],\"Right\":[{\"id\":\"N2\",\"label\":\"~2\",\"type\":\"foundation.electrical.three_phase\"}],\"Top\":[{\"id\":\"Pm\",\"label\":\"P\",\"type\":\"output\"},{\"id\":\"Qm\",\"label\":\"Q\",\"type\":\"output\"}]}"
  Real-Imag to Complex : RealImagToComplex
  Real-Imag to Complex1 : RealImagToComplex
  current_voltage : ee_lib/Sensors & Transducers/Current and Voltage Sensor (Three-Phase)  vMeasurementType=ee.enum.vmeasurement.lg  outputUnit=ee.enum.unit.pu  SRated=Pnom A*V  VRated=Vnom V  I_specify=off  I_priority=None  I=[0, 0, 0] A  I_nominal_specify=off  I_nominal_value=1  I_nominal_unit=A  V_specify=off  V_priority=None  V=[0, 0, 0] V  V_nominal_specify=off  V_nominal_value=1  V_nominal_unit=V
      settings: InternalSimscapePortConfiguration="{\"Bottom\":[],\"Left\":[{\"id\":\"N1\",\"label\":\"~1\",\"type\":\"foundation.electrical.three_phase\"}],\"Right\":[{\"id\":\"V_output\",\"label\":\"V\",\"type\":\"output\"},{\"id\":\"I_output\",\"label\":\"I\",\"type\":\"output\"},{\"id\":\"N2\",\"label\":\"~2\",\"type\":\"foundation.electrical.three_phase\"}],\"Top\":[]}"
  ~1 : PMIOPort  Side=Left
  ~2 : PMIOPort  Port=2  Side=Right
  tag scope: Iabc_Gen=global, P_W=global, Q_var=global, Vabc_Gen=global
  wires:
  PS-Simulink Converter1/1 -> Real-Imag to Complex/2
  PS-Simulink Converter/1 -> Real-Imag to Complex/1
  Real-Imag to Complex/1 -> [Vabc_Gen]
  PS-Simulink Converter2/1 -> Real-Imag to Complex1/1
  PS-Simulink Converter3/1 -> Real-Imag to Complex1/2
  Real-Imag to Complex1/1 -> [Iabc_Gen]
  PS-Simulink Converter5/1 -> [P_W]
  PS-Simulink Converter4/1 -> [Q_var]
  connections:
  current_voltage/RConn3 -- ~1/RConn1
  Power Sensor (Three-Phase)/LConn1 -- current_voltage/LConn1
  "PS Harmonic Estimator (Real, Imaginary) V"/LConn1 -- current_voltage/RConn1
  "PS Harmonic Estimator (Real, Imaginary) I"/LConn1 -- current_voltage/RConn2
  PS-Simulink Converter/LConn1 -- "PS Harmonic Estimator (Real, Imaginary) V"/RConn1
  PS-Simulink Converter1/LConn1 -- "PS Harmonic Estimator (Real, Imaginary) V"/RConn2
  "PS Harmonic Estimator (Real, Imaginary) I"/RConn2 -- PS-Simulink Converter3/LConn1
  "PS Harmonic Estimator (Real, Imaginary) I"/RConn1 -- PS-Simulink Converter2/LConn1
  ~2/RConn1 -- Power Sensor (Three-Phase)/RConn1
  PS-Simulink Converter4/LConn1 -- Power Sensor (Three-Phase)/LConn3
  PS-Simulink Converter5/LConn1 -- Power Sensor (Three-Phase)/LConn2

== system Generator_Lib/Full/Flexible Shaft Network Coupler ==
  note: Connect Port 1 to the network
      | with the smaller sample time, or
      | the network running variable step.
  note: Uncomment rate transition
      | blocks if one or both networks
      | are running fixed step.
  Port 1 Interface : Subsystem  mask(Network Coupler (Flexible Shaft) Port 1 Interface){interfaceModel=an actual shaft compliance, k=25000, lambda=200, samplingType=Variable step at ports 1 and 2, ts=0.001, h1=0.001, h2=0.01, predictionDiscreteToContinuous=off, smoothingContinuousToDiscrete=off, predictionSlowToFast=off, smoothingFastToSlow=off, nSmooth=1, tsSmoothing=0.01, J1=1, J2=1, tsRecommended=0.0026611, hRecommended=0.00026611, kDerived=250, lambdaDerived=20, tsMax=0.11975, through0=0}
      mask prompts: interfaceModel "physmod:simscape:couplers:SimscapeNetworkCouplersLib:SeparateUsing_MP"; k "physmod:simscape:couplers:SimscapeNetworkCouplersLib:ShaftStiffnessNmrad_MP"; lambda "physmod:simscape:couplers:SimscapeNetworkCouplersLib:ShaftDampingNmrads_MP"; samplingType "physmod:simscape:couplers:SimscapeNetworkCouplersLib:SamplingType_MP"; ts "physmod:simscape:couplers:SimscapeNetworkCouplersLib:SeparatorTimeConstants_MP"; h1 "physmod:simscape:couplers:SimscapeNetworkCouplersLib:Port1NetworkDiscreteSampleTimes_MP"; h2 "physmod:simscape:couplers:SimscapeNetworkCouplersLib:Port2NetworkDiscreteSampleTimes_MP"; predictionDiscreteToContinuous "physmod:simscape:couplers:SimscapeNetworkCouplersLib:UsePredictionWhenConnectingFixedStepToVariableStep_MP"; smoothingContinuousToDiscrete "physmod:simscape:couplers:SimscapeNetworkCouplersLib:UseSmoothingWhenConnectingVariableStepToFixedStep_MP"; predictionSlowToFast "physmod:simscape:couplers:SimscapeNetworkCouplersLib:UsePredictionWhenConnectingSlowToFastSampleTimes_MP"; smoothingFastToSlow "physmod:simscape:couplers:SimscapeNetworkCouplersLib:UseSmoothingWhenConnectingFastToSlowSampleTimes_MP"; nSmooth "physmod:simscape:couplers:SimscapeNetworkCouplersLib:NumberOfSamplesOverWhichToSmooth_MP"; tsSmoothing "physmod:simscape:couplers:SimscapeNetworkCouplersLib:SmoothingTimeConstants_MP"; J1 "physmod:simscape:couplers:SimscapeNetworkCouplersLib:ApproximateInertiaAtPort1kgm2_MP"; J2 "physmod:simscape:couplers:SimscapeNetworkCouplersLib:ApproximateInertiaAtPort2kgm2_MP"; tsRecommended "physmod:simscape:couplers:SimscapeNetworkCouplersLib:RecommendedMaxFilterTimeConstants_MP"; hRecommended "physmod:simscape:couplers:SimscapeNetworkCouplersLib:RecommendedMaxDiscreteSampleTimes_MP"; kDerived "physmod:simscape:couplers:SimscapeNetworkCouplersLib:CalculatedShaftStiffnessNmrad_MP"; lambdaDerived "physmod:simscape:couplers:SimscapeNetworkCouplersLib:CalculatedShaftDampingNmrads_MP"; tsMax "physmod:simscape:couplers:SimscapeNetworkCouplersLib:CalculatedFastestTrackableTimeConstants_MP"; through0 "physmod:simscape:couplers:SimscapeNetworkCouplersLib:InitialTransmittedTorqueNm_MP"
      mask help: physmod:simscape:couplers:SimscapeNetworkCouplersLib:NetworkCouplerFlexibleShaftPort1Interface_MD
      mask init:
      | % Fixed step sample time value check
      | foundation.internal.couplers.checkSampleTimes(gcb,h1,h2);
      | 
      | % Map mask choices to Simscape block parameters  
      | [K,Lambda,tau,~,~,x0,~] = foundation.internal.couplers.mechanical.derivedParamsRotational(...
      |     gcb,ts,h1,h2,through0,k,lambda,J1,J2);
      settings: PortSchema="{\"entries\":[{\"content\":{\"sides\":[{\"content\":{\"connectorIds\":[\"LConn1\"]},\"type\":\"ConnectorPlacement.EquallySpacedRectSide\",\"uuid\":\"a6d4a9fd-b5aa-40dc-ab7e-2b646b9b57bc\"},{\"content\":{\"connectorIds\":[\"Out1\",\"In1\"],\"side\":\"RIGHT\"},\"type\":\"ConnectorPlacement.EquallySpacedRectSide\",\"uuid\":\"31bb6273-5b9b-48d0-a1a2-6fbacb979b97\"},{\"content\":{\"connectorIds\":[],\"side\":\"TOP\"},\"type\":\"ConnectorPlacement.EquallySpacedRectSide\",\"uuid\":\"0f7afab2-4481-486c-9ad0-2b42c5b091a4\"}]},\"type\":\"ConnectorPlacement.EquallySpacedConnector\",\"uuid\":\"a98e47aa-cbfd-441a-b14c-c9ea515c056e\"}],\"packageUris\":[\"http://schema.mathworks.com/mf0/Connector/R2020b\"],\"version\":\"1.0\"}"
      mask Help: web([docroot '/simscape/ref/networkcouplerflexibleshaft.html'])
      mask TypeOptions interfaceModel: physmod:simscape:couplers:SimscapeNetworkCouplersLib:anActualShaftCompliance_PV | physmod:simscape:couplers:SimscapeNetworkCouplersLib:anAddedNumericalCompliance_PV
      mask Callback interfaceModel: foundation.internal.couplers.mechanical.parameterVisibilities(gcb)
      mask TypeOptions samplingType: physmod:simscape:couplers:SimscapeNetworkCouplersLib:VariableStepAtPorts1And2_PV | physmod:simscape:couplers:SimscapeNetworkCouplersLib:VariableStepAtPort1AndFixedStepAtPort2_PV | physmod:simscape:couplers:SimscapeNetworkCouplersLib:FixedStepBothPortsWithCommonSampleTime_PV | physmod:simscape:couplers:SimscapeNetworkCouplersLib:FixedStepBothPortsWithFasterSamplingAtPort1_PV
      mask Callback samplingType: foundation.internal.couplers.mechanical.parameterVisibilities(gcb)
      mask Callback predictionDiscreteToContinuous: foundation.internal.couplers.mechanical.parameterVisibilities(gcb)
      mask Callback smoothingContinuousToDiscrete: foundation.internal.couplers.mechanical.parameterVisibilities(gcb)
      mask Callback predictionSlowToFast: foundation.internal.couplers.mechanical.parameterVisibilities(gcb)
      mask Callback smoothingFastToSlow: foundation.internal.couplers.mechanical.parameterVisibilities(gcb)
      mask DialogControl Main Prompt: physmod:simscape:couplers:SimscapeNetworkCouplersLib:tab_Main
      mask DialogControl interfaceModel Prompt: Separate using
      mask DialogControl k Prompt: Shaft stiffness (Nm/rad)
      mask DialogControl lambda Prompt: Shaft damping (Nm/(rad/s))
      mask DialogControl samplingType Prompt: Sampling type
      mask DialogControl ts Prompt: Separator time constant (s)
      mask DialogControl h1 Prompt: Port 1 network discrete sample time (s)
      mask DialogControl h2 Prompt: Port 2 network discrete sample time (s)
      mask DialogControl predictionDiscreteToContinuous Prompt: Use prediction when connecting fixed step to variable step
      mask DialogControl smoothingContinuousToDiscrete Prompt: Use smoothing when connecting variable step to fixed step
      mask DialogControl predictionSlowToFast Prompt: Use prediction when connecting slow to fast sample times
      mask DialogControl smoothingFastToSlow Prompt: Use smoothing when connecting fast to slow sample times
      mask DialogControl nSmooth Prompt: Number of samples over which to smooth
      mask DialogControl tsSmoothing Prompt: Smoothing time constant (s)
      mask DialogControl Analysis Prompt: physmod:simscape:couplers:SimscapeNetworkCouplersLib:tab_Analysis
      mask DialogControl connectedNetworkInfo Prompt: physmod:simscape:couplers:SimscapeNetworkCouplersLib:heading_ConnectedNetworkInformation
      mask DialogControl J1 Prompt: Approximate inertia at port 1 (kg*m^2)
      mask DialogControl J2 Prompt: Approximate inertia at port 2 (kg*m^2)
      mask DialogControl derivedValues Prompt: physmod:simscape:couplers:SimscapeNetworkCouplersLib:heading_DerivedValues
      mask DialogControl tsRecommended Prompt: Recommended max filter time constant (s)
      mask DialogControl hRecommended Prompt: Recommended max discrete sample time (s)
      mask DialogControl kDerived Prompt: Calculated shaft stiffness (Nm/rad)
      mask DialogControl lambdaDerived Prompt: Calculated shaft damping (Nm/(rad/s))
      mask DialogControl tsMax Prompt: Calculated fastest trackable time constant (s)
      mask DialogControl updateRecommendations Prompt: physmod:simscape:couplers:SimscapeNetworkCouplersLib:button_Update
      mask DialogControl updateRecommendations Callback: foundation.internal.couplers.mechanical.analysisRotational(gcb);
      mask DialogControl InitialConditions Prompt: physmod:simscape:couplers:SimscapeNetworkCouplersLib:tab_InitialConditions
      mask DialogControl through0 Prompt: Initial transmitted torque (Nm)
  Port 2 Interface : Subsystem  mask(Network Coupler (Flexible Shaft) Port 2 Interface){}
      mask help: physmod:simscape:couplers:SimscapeNetworkCouplersLib:NetworkCouplerFlexibleShaftPort2Interface_MD
      settings: PortSchema="{\"entries\":[{\"content\":{\"sides\":[{\"content\":{\"connectorIds\":[\"In1\",\"Out1\"]},\"type\":\"ConnectorPlacement.EquallySpacedRectSide\",\"uuid\":\"5a4c1550-e77d-42df-bf3e-b81963920de7\"},{\"content\":{\"connectorIds\":[\"RConn1\"],\"side\":\"RIGHT\"},\"type\":\"ConnectorPlacement.EquallySpacedRectSide\",\"uuid\":\"3fd730f7-5937-4563-a365-595aaae9027b\"},{\"content\":{\"connectorIds\":[],\"side\":\"TOP\"},\"type\":\"ConnectorPlacement.EquallySpacedRectSide\",\"uuid\":\"c16e04e4-26e8-4fd6-98d3-59adbef44c0d\"}]},\"type\":\"ConnectorPlacement.EquallySpacedConnector\",\"uuid\":\"5588d8d0-d459-45fe-a303-1ca6654e99d0\"}],\"packageUris\":[\"http://schema.mathworks.com/mf0/Connector/R2020b\"],\"version\":\"1.0\"}"
      mask Help: web([docroot '/simscape/ref/networkcouplerflexibleshaft.html'])
  Rate transition (fast-to-slow) : RateTransition  Commented=through  Integrity=off
  Rate transition (slow-to-fast) : RateTransition  Commented=through  Integrity=off
  1 : PMIOPort  Side=Left
  2 : PMIOPort  Port=2  Side=Right
  wires:
  Rate transition (slow-to-fast)/1 -> Port 1 Interface/1(speed)
  Port 2 Interface/1(speed) -> Rate transition (slow-to-fast)/1
  Rate transition (fast-to-slow)/1 -> Port 2 Interface/1(torque)
  Port 1 Interface/1(torque) -> Rate transition (fast-to-slow)/1
  connections:
  1/RConn1 -- Port 1 Interface/LConn1
  2/RConn1 -- Port 2 Interface/RConn1
